simulink model "MMC_phase_discentralized_HAAS_20260927"  (R2024b)
settings: Solver=FixedStepDiscrete  StartTime=t_init_sim  StopTime=sim_time  FixedStep=Ts  RelTol=1e-3
values from neighbouring files (symbols this model uses):
  a = 1    [script_MMC_phase_hackathon_NLM_discentralized_HAAS_20260927.m]
  C1low1_active = 1    [script_MMC_phase_hackathon_NLM_discentralized_HAAS_20260927.m]
  C2low1_active = 1    [script_MMC_phase_hackathon_NLM_discentralized_HAAS_20260927.m]
  C_bus = 4400e-6    (= 0.0044)    [script_MMC_phase_hackathon_NLM_discentralized_HAAS_20260927.m]
  C_M_extra = C_m-twist_high_side_C    [script_MMC_phase_hackathon_NLM_discentralized_HAAS_20260927.m]
  duty_cycle = 1.0    (= 1)    [script_MMC_phase_hackathon_NLM_discentralized_HAAS_20260927.m]
  f0 = 50    [script_MMC_phase_hackathon_NLM_discentralized_HAAS_20260927.m]
  feeder_current_lower_rate_limit = -10    [script_MMC_phase_hackathon_NLM_discentralized_HAAS_20260927.m]    (also in twist_parameters.m = -500)
  feeder_current_tab = [0.328 0.217 0.162 0.132 0.109 0.094 0.083 0.075 0.068 0.062 0.058 0.054 ... (42 elements, 14x3)]    [feeder_current.mat]
  feeder_current_upper_rate_limit = 0.386/(20e-3)    (= 19.3)    [twist_parameters.m]
  is6VExternallySupplied = true    [script_MMC_phase_hackathon_NLM_discentralized_HAAS_20260927.m]
  isFeederJumperOpen = true    [script_MMC_phase_hackathon_NLM_discentralized_HAAS_20260927.m]
  L_arm = 30e-3    (= 0.03)    [script_MMC_phase_hackathon_NLM_discentralized_HAAS_20260927.m]
  m = 1    [script_MMC_phase_hackathon_NLM_discentralized_HAAS_20260927.m]
  N = 5    [script_MMC_phase_hackathon_NLM_discentralized_HAAS_20260927.m]
  power_losses = false    [script_MMC_phase_hackathon_NLM_discentralized_HAAS_20260927.m]
  R = 15    [script_MMC_phase_hackathon_NLM_discentralized_HAAS_20260927.m]
  R_arm = 0.2    [script_MMC_phase_hackathon_NLM_discentralized_HAAS_20260927.m]
  source_V = 0    [script_MMC_phase_hackathon_NLM_discentralized_HAAS_20260927.m]
  Tcom_sample = round(Tcom / Ts)    [script_MMC_phase_hackathon_NLM_discentralized_HAAS_20260927.m]
  time_charge = 0.1    [script_MMC_phase_hackathon_NLM_discentralized_HAAS_20260927.m]
  time_decharge = 1.5    [script_MMC_phase_hackathon_NLM_discentralized_HAAS_20260927.m]
  Ts = 1e-6    (= 1e-06)    [script_MMC_phase_hackathon_NLM_discentralized_HAAS_20260927.m]
  twist_data_acquisition_delay = 50e-9    (= 5e-08)    [script_MMC_phase_hackathon_NLM_discentralized_HAAS_20260927.m]    (also in twist_parameters.m)
  twist_data_sampling_period = 1/twist_freq_data_sampling    (= 5e-05)    [script_MMC_phase_hackathon_NLM_discentralized_HAAS_20260927.m]    (also in twist_parameters.m)
  twist_dead_time = 200e-9    (= 2e-07)    [twist_parameters.m]
  twist_freq_switching = 200e3    (= 200000)    [twist_parameters.m]
  twist_high_side_adc_R = 1/(1/2e6 + 1/2e6 + 1/(330e3+5.6e3))    (= 251272.836178)    [twist_parameters.m]
  twist_high_side_C = 33e-6*4 + 4.7e-6*12    (= 0.0001884)    [twist_parameters.m]
  twist_high_side_feeder_R = 47e3+4.7e3    (= 51700)    [twist_parameters.m]
  twist_high_side_rC = 0.1    [twist_parameters.m]
  twist_low_side_adc_R = 150e3+470    (= 150470)    [twist_parameters.m]
  twist_low_side_C_ceramic = 3*4.7e-6    (= 1.41e-05)    [twist_parameters.m]
  twist_low_side_C_electrolytic = 47e-6    (= 4.7e-05)    [twist_parameters.m]
  twist_low_side_L = 33e-6    (= 3.3e-05)    [twist_parameters.m]
  twist_low_side_rC = 700e-3    (= 0.7)    [twist_parameters.m]
  twist_low_side_rL = 20e-3    (= 0.02)    [twist_parameters.m]
  twist_R_VCC = (tau_VCC/twist_high_side_C  - twist_high_side_rC)/(1-(tau_VCC/twist_high_side_C - twist_high_side_rC)/R_parallel)    (= 1110.74997822)    [twist_parameters.m]
  VDC = 48    [script_MMC_phase_hackathon_NLM_discentralized_HAAS_20260927.m]
undefined symbols (not defined in the file or in its folder): C_SM, feeder_current, gcbh, sps_rtmsupport, twist_low_side_lC
libraries: spsSeriesRLCBranchLib x135, spsTriangleGeneratorLib x60, spsMosfetLib x60, spsCurrentMeasurementLib x43, spsVoltageMeasurementLib x35, spsControlledCurrentSourceLib x30, spsDiodeLib x22, spsIdealSwitchLib x20, spsControlledVoltageSourceLib x1, spsGroundLib x1, spspowerguiLib x1
(part 2 of 22)

== system MMC_phase_discentralized_HAAS_20260927/ /Communication_subsystem/Lower_arm ==
  sync : Inport
  lower_arm_info : Inport  Port=2
  M6_RX_signal : Inport  Port=3
  M7_RX_signal : Inport  Port=4
  M8_RX_signal : Inport  Port=5
  M9_RX_signal : Inport  Port=6
  M10_RX_signal : Inport  Port=7
  M1_Comm : Subsystem
      settings: PortSchema="{\"entries\":[{\"content\":{\"sides\":[{\"content\":{\"connectorIds\":[\"In1\",\"Out2\"]},\"type\":\"ConnectorPlacement.EquallySpacedRectSide\",\"uuid\":\"47077a1e-eba1-4129-8203-93262b2de465\"},{\"content\":{\"connectorIds\":[\"Out1\",\"In3\"],\"side\":\"RIGHT\"},\"type\":\"ConnectorPlacement.EquallySpacedRectSide\",\"uuid\":\"701fdbad-c928-45f3-8ba2-a14f680316f8\"},{\"content\":{\"side\":\"TOP\"},\"type\":\"ConnectorPlacement.EquallySpacedRectSide\",\"uuid\":\"d648951b-caea-4569-a411-8455254fdbc0\"},{\"content\":{\"connectorIds\":[\"In2\"],\"side\":\"BOTTOM\"},\"type\":\"ConnectorPlacement.EquallySpacedRectSide\",\"uuid\":\"07eb9aa1-f407-41f0-8942-d6ed405114b5\"}]},\"type\":\"ConnectorPlacement.EquallySpacedConnector\",\"uuid\":\"7c33ff72-602e-419f-9c2d-5eefc0d60400\"}],\"packageUris\":[\"http://schema.mathworks.com/mf0/Connector/R2020b\"],\"version\":\"1.0\"}"
  M2_Comm : Subsystem
      settings: PortSchema="{\"entries\":[{\"content\":{\"sides\":[{\"content\":{\"connectorIds\":[\"In1\",\"Out2\"]},\"type\":\"ConnectorPlacement.EquallySpacedRectSide\",\"uuid\":\"47077a1e-eba1-4129-8203-93262b2de465\"},{\"content\":{\"connectorIds\":[\"Out1\",\"In3\"],\"side\":\"RIGHT\"},\"type\":\"ConnectorPlacement.EquallySpacedRectSide\",\"uuid\":\"701fdbad-c928-45f3-8ba2-a14f680316f8\"},{\"content\":{\"side\":\"TOP\"},\"type\":\"ConnectorPlacement.EquallySpacedRectSide\",\"uuid\":\"d648951b-caea-4569-a411-8455254fdbc0\"},{\"content\":{\"connectorIds\":[\"In2\"],\"side\":\"BOTTOM\"},\"type\":\"ConnectorPlacement.EquallySpacedRectSide\",\"uuid\":\"01601a56-4c3c-4c18-be21-822f443ca232\"}]},\"type\":\"ConnectorPlacement.EquallySpacedConnector\",\"uuid\":\"7c33ff72-602e-419f-9c2d-5eefc0d60400\"}],\"packageUris\":[\"http://schema.mathworks.com/mf0/Connector/R2020b\"],\"version\":\"1.0\"}"
  M3_Comm : Subsystem
      settings: PortSchema="{\"entries\":[{\"content\":{\"sides\":[{\"content\":{\"connectorIds\":[\"In1\",\"Out2\"]},\"type\":\"ConnectorPlacement.EquallySpacedRectSide\",\"uuid\":\"47077a1e-eba1-4129-8203-93262b2de465\"},{\"content\":{\"connectorIds\":[\"Out1\",\"In3\"],\"side\":\"RIGHT\"},\"type\":\"ConnectorPlacement.EquallySpacedRectSide\",\"uuid\":\"701fdbad-c928-45f3-8ba2-a14f680316f8\"},{\"content\":{\"side\":\"TOP\"},\"type\":\"ConnectorPlacement.EquallySpacedRectSide\",\"uuid\":\"d648951b-caea-4569-a411-8455254fdbc0\"},{\"content\":{\"connectorIds\":[\"In2\"],\"side\":\"BOTTOM\"},\"type\":\"ConnectorPlacement.EquallySpacedRectSide\",\"uuid\":\"b7518228-bb66-4696-b5d4-126a1140e1c3\"}]},\"type\":\"ConnectorPlacement.EquallySpacedConnector\",\"uuid\":\"7c33ff72-602e-419f-9c2d-5eefc0d60400\"}],\"packageUris\":[\"http://schema.mathworks.com/mf0/Connector/R2020b\"],\"version\":\"1.0\"}"
  M4_Comm : Subsystem
      settings: PortSchema="{\"entries\":[{\"content\":{\"sides\":[{\"content\":{\"connectorIds\":[\"In1\",\"Out2\"]},\"type\":\"ConnectorPlacement.EquallySpacedRectSide\",\"uuid\":\"47077a1e-eba1-4129-8203-93262b2de465\"},{\"content\":{\"connectorIds\":[\"Out1\",\"In3\"],\"side\":\"RIGHT\"},\"type\":\"ConnectorPlacement.EquallySpacedRectSide\",\"uuid\":\"701fdbad-c928-45f3-8ba2-a14f680316f8\"},{\"content\":{\"side\":\"TOP\"},\"type\":\"ConnectorPlacement.EquallySpacedRectSide\",\"uuid\":\"d648951b-caea-4569-a411-8455254fdbc0\"},{\"content\":{\"connectorIds\":[\"In2\"],\"side\":\"BOTTOM\"},\"type\":\"ConnectorPlacement.EquallySpacedRectSide\",\"uuid\":\"5f4b38d1-ea61-4297-b8b6-4cb7ffcc6410\"}]},\"type\":\"ConnectorPlacement.EquallySpacedConnector\",\"uuid\":\"7c33ff72-602e-419f-9c2d-5eefc0d60400\"}],\"packageUris\":[\"http://schema.mathworks.com/mf0/Connector/R2020b\"],\"version\":\"1.0\"}"
  M5_Comm : Subsystem
      settings: PortSchema="{\"entries\":[{\"content\":{\"sides\":[{\"content\":{\"connectorIds\":[\"In1\",\"Out2\"]},\"type\":\"ConnectorPlacement.EquallySpacedRectSide\",\"uuid\":\"47077a1e-eba1-4129-8203-93262b2de465\"},{\"content\":{\"connectorIds\":[\"Out1\",\"In3\"],\"side\":\"RIGHT\"},\"type\":\"ConnectorPlacement.EquallySpacedRectSide\",\"uuid\":\"701fdbad-c928-45f3-8ba2-a14f680316f8\"},{\"content\":{\"side\":\"TOP\"},\"type\":\"ConnectorPlacement.EquallySpacedRectSide\",\"uuid\":\"d648951b-caea-4569-a411-8455254fdbc0\"},{\"content\":{\"connectorIds\":[\"In2\"],\"side\":\"BOTTOM\"},\"type\":\"ConnectorPlacement.EquallySpacedRectSide\",\"uuid\":\"cd08f752-2006-4da0-88d6-bb4b20ac3ab7\"}]},\"type\":\"ConnectorPlacement.EquallySpacedConnector\",\"uuid\":\"7c33ff72-602e-419f-9c2d-5eefc0d60400\"}],\"packageUris\":[\"http://schema.mathworks.com/mf0/Connector/R2020b\"],\"version\":\"1.0\"}"
  M6_TX_signal : Outport
  M7_TX_signal : Outport  Port=2
  M8_TX_signal : Outport  Port=3
  M9_TX_signal : Outport  Port=4
  M10_TX_signal : Outport  Port=5
  wires:
  [lower_arm_info] -> M5_Comm/1(TX_variables)
  M4_Comm/1(TX_signal) -> M9_TX_signal/1
  [lower_arm_info] -> M1_Comm/1(TX_variables)
  [lower_arm_info] -> M4_Comm/1(TX_variables)
  M3_Comm/1(TX_signal) -> M8_TX_signal/1
  M2_Comm/1(TX_signal) -> M7_TX_signal/1
  [lower_arm_info] -> M2_Comm/1(TX_variables)
  [lower_arm_info] -> M3_Comm/1(TX_variables)
  M6_RX_signal/1 -> M1_Comm/3(RX_signal)
  [sync] -> M3_Comm/2(sync)
  M8_RX_signal/1 -> M3_Comm/3(RX_signal)
  [sync] -> M5_Comm/2(sync)
  [sync] -> M4_Comm/2(sync)
  [sync] -> M1_Comm/2(sync)
  M10_RX_signal/1 -> M5_Comm/3(RX_signal)
  M1_Comm/1(TX_signal) -> M6_TX_signal/1
  M7_RX_signal/1 -> M2_Comm/3(RX_signal)
  [sync] -> M2_Comm/2(sync)
  M5_Comm/1(TX_signal) -> M10_TX_signal/1
  M9_RX_signal/1 -> M4_Comm/3(RX_signal)
  lower_arm_info/1 -> [lower_arm_info]
  sync/1 -> [sync]

== system MMC_phase_discentralized_HAAS_20260927/ /Communication_subsystem/Upper_arm ==
  upper_arm_info : Inport
  sync : Inport  Port=2
  M1_RX_signal : Inport  Port=3
  M2_RX_signal : Inport  Port=4
  M3_RX_signal : Inport  Port=5
  M4_RX_signal : Inport  Port=6
  M5_RX_signal : Inport  Port=7
  M1_Comm : Subsystem
      settings: PortSchema="{\"entries\":[{\"content\":{\"sides\":[{\"content\":{\"connectorIds\":[\"In1\",\"Out2\"]},\"type\":\"ConnectorPlacement.EquallySpacedRectSide\",\"uuid\":\"c3733cfa-9814-4ae5-a55a-8e5b6f8a57d7\"},{\"content\":{\"connectorIds\":[\"Out1\",\"In3\"],\"side\":\"RIGHT\"},\"type\":\"ConnectorPlacement.EquallySpacedRectSide\",\"uuid\":\"d16535d3-81ee-4162-a646-15cef1f1639a\"},{\"content\":{\"side\":\"TOP\"},\"type\":\"ConnectorPlacement.EquallySpacedRectSide\",\"uuid\":\"672d53ef-99b6-4fa6-8351-42251f607454\"},{\"content\":{\"connectorIds\":[\"In2\"],\"side\":\"BOTTOM\"},\"type\":\"ConnectorPlacement.EquallySpacedRectSide\",\"uuid\":\"a9bd7512-44c2-4af9-8132-4c17be33b3c2\"}]},\"type\":\"ConnectorPlacement.EquallySpacedConnector\",\"uuid\":\"554aea8b-7fd0-4035-ac75-3acab423d605\"}],\"packageUris\":[\"http://schema.mathworks.com/mf0/Connector/R2020b\"],\"version\":\"1.0\"}"
  M2_Comm : Subsystem
      settings: PortSchema="{\"entries\":[{\"content\":{\"sides\":[{\"content\":{\"connectorIds\":[\"In1\",\"Out2\"]},\"type\":\"ConnectorPlacement.EquallySpacedRectSide\",\"uuid\":\"47077a1e-eba1-4129-8203-93262b2de465\"},{\"content\":{\"connectorIds\":[\"Out1\",\"In3\"],\"side\":\"RIGHT\"},\"type\":\"ConnectorPlacement.EquallySpacedRectSide\",\"uuid\":\"701fdbad-c928-45f3-8ba2-a14f680316f8\"},{\"content\":{\"side\":\"TOP\"},\"type\":\"ConnectorPlacement.EquallySpacedRectSide\",\"uuid\":\"d648951b-caea-4569-a411-8455254fdbc0\"},{\"content\":{\"connectorIds\":[\"In2\"],\"side\":\"BOTTOM\"},\"type\":\"ConnectorPlacement.EquallySpacedRectSide\",\"uuid\":\"d4b1d2d6-b4a1-4e2c-9ca6-248db102ef7c\"}]},\"type\":\"ConnectorPlacement.EquallySpacedConnector\",\"uuid\":\"7c33ff72-602e-419f-9c2d-5eefc0d60400\"}],\"packageUris\":[\"http://schema.mathworks.com/mf0/Connector/R2020b\"],\"version\":\"1.0\"}"
  M3_Comm : Subsystem
      settings: PortSchema="{\"entries\":[{\"content\":{\"sides\":[{\"content\":{\"connectorIds\":[\"In1\",\"Out2\"]},\"type\":\"ConnectorPlacement.EquallySpacedRectSide\",\"uuid\":\"47077a1e-eba1-4129-8203-93262b2de465\"},{\"content\":{\"connectorIds\":[\"Out1\",\"In3\"],\"side\":\"RIGHT\"},\"type\":\"ConnectorPlacement.EquallySpacedRectSide\",\"uuid\":\"701fdbad-c928-45f3-8ba2-a14f680316f8\"},{\"content\":{\"side\":\"TOP\"},\"type\":\"ConnectorPlacement.EquallySpacedRectSide\",\"uuid\":\"d648951b-caea-4569-a411-8455254fdbc0\"},{\"content\":{\"connectorIds\":[\"In2\"],\"side\":\"BOTTOM\"},\"type\":\"ConnectorPlacement.EquallySpacedRectSide\",\"uuid\":\"e45915a7-b7a2-4a5e-b9ff-be90cdaaaa95\"}]},\"type\":\"ConnectorPlacement.EquallySpacedConnector\",\"uuid\":\"7c33ff72-602e-419f-9c2d-5eefc0d60400\"}],\"packageUris\":[\"http://schema.mathworks.com/mf0/Connector/R2020b\"],\"version\":\"1.0\"}"
  M4_Comm : Subsystem
      settings: PortSchema="{\"entries\":[{\"content\":{\"sides\":[{\"content\":{\"connectorIds\":[\"In1\",\"Out2\"]},\"type\":\"ConnectorPlacement.EquallySpacedRectSide\",\"uuid\":\"47077a1e-eba1-4129-8203-93262b2de465\"},{\"content\":{\"connectorIds\":[\"Out1\",\"In3\"],\"side\":\"RIGHT\"},\"type\":\"ConnectorPlacement.EquallySpacedRectSide\",\"uuid\":\"701fdbad-c928-45f3-8ba2-a14f680316f8\"},{\"content\":{\"side\":\"TOP\"},\"type\":\"ConnectorPlacement.EquallySpacedRectSide\",\"uuid\":\"d648951b-caea-4569-a411-8455254fdbc0\"},{\"content\":{\"connectorIds\":[\"In2\"],\"side\":\"BOTTOM\"},\"type\":\"ConnectorPlacement.EquallySpacedRectSide\",\"uuid\":\"fe4854bf-7531-4052-9f9a-05b48e3d1945\"}]},\"type\":\"ConnectorPlacement.EquallySpacedConnector\",\"uuid\":\"7c33ff72-602e-419f-9c2d-5eefc0d60400\"}],\"packageUris\":[\"http://schema.mathworks.com/mf0/Connector/R2020b\"],\"version\":\"1.0\"}"
  M5_Comm : Subsystem
      settings: PortSchema="{\"entries\":[{\"content\":{\"sides\":[{\"content\":{\"connectorIds\":[\"In1\",\"Out2\"]},\"type\":\"ConnectorPlacement.EquallySpacedRectSide\",\"uuid\":\"47077a1e-eba1-4129-8203-93262b2de465\"},{\"content\":{\"connectorIds\":[\"Out1\",\"In3\"],\"side\":\"RIGHT\"},\"type\":\"ConnectorPlacement.EquallySpacedRectSide\",\"uuid\":\"701fdbad-c928-45f3-8ba2-a14f680316f8\"},{\"content\":{\"side\":\"TOP\"},\"type\":\"ConnectorPlacement.EquallySpacedRectSide\",\"uuid\":\"d648951b-caea-4569-a411-8455254fdbc0\"},{\"content\":{\"connectorIds\":[\"In2\"],\"side\":\"BOTTOM\"},\"type\":\"ConnectorPlacement.EquallySpacedRectSide\",\"uuid\":\"76d1056e-e7b2-4023-89b8-57825a028de1\"}]},\"type\":\"ConnectorPlacement.EquallySpacedConnector\",\"uuid\":\"7c33ff72-602e-419f-9c2d-5eefc0d60400\"}],\"packageUris\":[\"http://schema.mathworks.com/mf0/Connector/R2020b\"],\"version\":\"1.0\"}"
  M1_TX_signal : Outport
  M2_TX_signal : Outport  Port=2
  M3_TX_signal : Outport  Port=3
  M4_TX_signal : Outport  Port=4
  M5_TX_signal : Outport  Port=5
  RX_Variables : Outport  Port=6
  wires:
  [upper_arm_info] -> M5_Comm/1(TX_variables)
  M4_Comm/1(TX_signal) -> M4_TX_signal/1
  [upper_arm_info] -> M1_Comm/1(TX_variables)
  [upper_arm_info] -> M4_Comm/1(TX_variables)
  M3_Comm/1(TX_signal) -> M3_TX_signal/1
  M2_Comm/1(TX_signal) -> M2_TX_signal/1
  [upper_arm_info] -> M2_Comm/1(TX_variables)
  [upper_arm_info] -> M3_Comm/1(TX_variables)
  M1_RX_signal/1 -> M1_Comm/3(RX_signal)
  [sync] -> M3_Comm/2(sync)
  M3_RX_signal/1 -> M3_Comm/3(RX_signal)
  [sync] -> M5_Comm/2(sync)
  [sync] -> M4_Comm/2(sync)
  [sync] -> M1_Comm/2(sync)
  M5_RX_signal/1 -> M5_Comm/3(RX_signal)
  M1_Comm/1(TX_signal) -> M1_TX_signal/1
  M2_RX_signal/1 -> M2_Comm/3(RX_signal)
  [sync] -> M2_Comm/2(sync)
  M5_Comm/1(TX_signal) -> M5_TX_signal/1
  M4_RX_signal/1 -> M4_Comm/3(RX_signal)
  upper_arm_info/1 -> [upper_arm_info]
  sync/1 -> [sync]
  M1_Comm/2(RX_Variables) -> RX_Variables/1

== system MMC_phase_discentralized_HAAS_20260927/ /Sinus Modulation + Sorting Algorithm/M1 MCU ==
  note: NLM
  note: NLM
  note: Modulation reference
  note: NLM modulation
  Vc_unitaire_stack : Inport
  i_stack : Inport  Port=2
  M_number : Inport  Port=3
  Pulse : Inport  Port=4
  CVB : MATLAB Function  TreatAsAtomicUnit=on
  Constant : Constant  Value=duty_cycle
  Constant4 : Constant  Value=a*1/2
  Gain : Gain  Gain=N
  Gain1 : Gain  Gain=m*1/2
  Gain2 : Gain  Gain=N
  Quantizer : Quantizer  QuantizationInterval=1
  Quantizer1 : Quantizer  QuantizationInterval=1
  Saturation : Saturate  UpperLimit=N  LowerLimit=0
  Saturation1 : Saturate  UpperLimit=N  LowerLimit=0
  Scope : Scope  NumInputPorts=5
  Sine Wave : Sin  Frequency=2*pi*f0  SampleTime=Ts
  Sorting : Subsystem
  Sum1 : Sum  Inputs=|+-
  Sum2 : Sum  Inputs=|++
  g_unitaire_stack : Outport
  N_u : Outport  Port=2
  N_l : Outport  Port=3
  tag scope: ml=global, mu=global
  wires:
  Vc_unitaire_stack/1 -> Sorting/1(Vc_u), Scope/1
  Sorting/1(Ordre_u) -> CVB/1(ordre)
  Saturation/1 -> N_u/1, Scope/4, CVB/3(N_on)
  i_stack/1 -> Scope/2, Sorting/2(i_u)
  Sorting/2(Sens_u) -> CVB/2(sens)
  Pulse/1 -> Scope/5, Sorting/Enable
  CVB/1(y) -> Scope/3, g_unitaire_stack/1
  Constant/1 -> CVB/4(duty_cycle)
  M_number/1 -> CVB/5(M_number)
  Gain/1 -> Quantizer/1
  Gain2/1 -> Quantizer1/1
  Constant4/1 -> Sum2/1, Sum1/1
  Gain1/1 -> Sum1/2, Sum2/2
  Sine Wave/1 -> Gain1/1
  Saturation1/1 -> N_l/1
  Quantizer1/1 -> Saturation1/1
  Sum1/1 -> Gain/1, [mu]
  Quantizer/1 -> Saturation/1
  Sum2/1 -> [ml], Gain2/1

== system MMC_phase_discentralized_HAAS_20260927/ /Sinus Modulation + Sorting Algorithm/M10 MCU ==
  Vc_unitaire_stack : Inport
  i_stack : Inport  Port=2
  N_on_stack : Inport  Port=3
  M_number : Inport  Port=4
  Pulse : Inport  Port=5
  CVB : MATLAB Function  TreatAsAtomicUnit=on
  Constant : Constant  Value=duty_cycle
  Scope : Scope  NumInputPorts=5
  Sorting : Subsystem
  g_unitaire_stack : Outport
  wires:
  Vc_unitaire_stack/1 -> Sorting/1(Vc_u), Scope/1
  Sorting/1(Ordre_u) -> CVB/1(ordre)
  N_on_stack/1 -> Scope/4, CVB/3(N_on)
  i_stack/1 -> Scope/2, Sorting/2(i_u)
  Sorting/2(Sens_u) -> CVB/2(sens)
  Pulse/1 -> Scope/5, Sorting/Enable
  CVB/1(y) -> Scope/3, g_unitaire_stack/1
  Constant/1 -> CVB/4(duty_cycle)
  M_number/1 -> CVB/5(M_number)

== system MMC_phase_discentralized_HAAS_20260927/ /Sinus Modulation + Sorting Algorithm/M2 MCU ==
  Vc_unitaire_stack : Inport
  i_stack : Inport  Port=2
  N_on_stack : Inport  Port=3
  M_number : Inport  Port=4
  Pulse : Inport  Port=5
  CVB : MATLAB Function  TreatAsAtomicUnit=on
  Constant : Constant  Value=duty_cycle
  Scope : Scope  NumInputPorts=5
  Sorting : Subsystem
  g_unitaire_stack : Outport
  wires:
  Vc_unitaire_stack/1 -> Sorting/1(Vc_u), Scope/1
  Sorting/1(Ordre_u) -> CVB/1(ordre)
  N_on_stack/1 -> Scope/4, CVB/3(N_on)
  i_stack/1 -> Scope/2, Sorting/2(i_u)
  Sorting/2(Sens_u) -> CVB/2(sens)
  Pulse/1 -> Scope/5, Sorting/Enable
  CVB/1(y) -> Scope/3, g_unitaire_stack/1
  Constant/1 -> CVB/4(duty_cycle)
  M_number/1 -> CVB/5(M_number)

== system MMC_phase_discentralized_HAAS_20260927/ /Sinus Modulation + Sorting Algorithm/M3 MCU ==
  Vc_unitaire_stack : Inport
  i_stack : Inport  Port=2
  N_on_stack : Inport  Port=3
  M_number : Inport  Port=4
  Pulse : Inport  Port=5
  CVB : MATLAB Function  TreatAsAtomicUnit=on
  Constant : Constant  Value=duty_cycle
  Scope : Scope  NumInputPorts=5
  Sorting : Subsystem
  g_unitaire_stack : Outport
  wires:
  Vc_unitaire_stack/1 -> Sorting/1(Vc_u), Scope/1
  Sorting/1(Ordre_u) -> CVB/1(ordre)
  N_on_stack/1 -> Scope/4, CVB/3(N_on)
  i_stack/1 -> Scope/2, Sorting/2(i_u)
  Sorting/2(Sens_u) -> CVB/2(sens)
  Pulse/1 -> Scope/5, Sorting/Enable
  CVB/1(y) -> Scope/3, g_unitaire_stack/1
  Constant/1 -> CVB/4(duty_cycle)
  M_number/1 -> CVB/5(M_number)

== system MMC_phase_discentralized_HAAS_20260927/ /Sinus Modulation + Sorting Algorithm/M4 MCU ==
  Vc_unitaire_stack : Inport
  i_stack : Inport  Port=2
  N_on_stack : Inport  Port=3
  M_number : Inport  Port=4
  Pulse : Inport  Port=5
  CVB : MATLAB Function  TreatAsAtomicUnit=on
  Constant : Constant  Value=duty_cycle
  Scope : Scope  NumInputPorts=5
  Sorting : Subsystem
  g_unitaire_stack : Outport
  wires:
  Vc_unitaire_stack/1 -> Sorting/1(Vc_u), Scope/1
  Sorting/1(Ordre_u) -> CVB/1(ordre)
  N_on_stack/1 -> Scope/4, CVB/3(N_on)
  i_stack/1 -> Scope/2, Sorting/2(i_u)
  Sorting/2(Sens_u) -> CVB/2(sens)
  Pulse/1 -> Scope/5, Sorting/Enable
  CVB/1(y) -> Scope/3, g_unitaire_stack/1
  Constant/1 -> CVB/4(duty_cycle)
  M_number/1 -> CVB/5(M_number)

== system MMC_phase_discentralized_HAAS_20260927/ /Sinus Modulation + Sorting Algorithm/M5 MCU ==
  Vc_unitaire_stack : Inport
  i_stack : Inport  Port=2
  N_on_stack : Inport  Port=3
  M_number : Inport  Port=4
  Pulse : Inport  Port=5
  CVB : MATLAB Function  TreatAsAtomicUnit=on
  Constant : Constant  Value=duty_cycle
  Scope : Scope  NumInputPorts=5
  Sorting : Subsystem
  g_unitaire_stack : Outport
  wires:
  Vc_unitaire_stack/1 -> Sorting/1(Vc_u), Scope/1
  Sorting/1(Ordre_u) -> CVB/1(ordre)
  N_on_stack/1 -> Scope/4, CVB/3(N_on)
  i_stack/1 -> Scope/2, Sorting/2(i_u)
  Sorting/2(Sens_u) -> CVB/2(sens)
  Pulse/1 -> Scope/5, Sorting/Enable
  CVB/1(y) -> Scope/3, g_unitaire_stack/1
  Constant/1 -> CVB/4(duty_cycle)
  M_number/1 -> CVB/5(M_number)

== system MMC_phase_discentralized_HAAS_20260927/ /Sinus Modulation + Sorting Algorithm/M6 MCU ==
  Vc_unitaire_stack : Inport
  i_stack : Inport  Port=2
  N_on_stack : Inport  Port=3
  M_number : Inport  Port=4
  Pulse : Inport  Port=5
  CVB : MATLAB Function  TreatAsAtomicUnit=on
  Constant : Constant  Value=duty_cycle
  Scope : Scope  NumInputPorts=5
  Sorting : Subsystem
  g_unitaire_stack : Outport
  wires:
  Vc_unitaire_stack/1 -> Sorting/1(Vc_u), Scope/1
  Sorting/1(Ordre_u) -> CVB/1(ordre)
  N_on_stack/1 -> Scope/4, CVB/3(N_on)
  i_stack/1 -> Scope/2, Sorting/2(i_u)
  Sorting/2(Sens_u) -> CVB/2(sens)
  Pulse/1 -> Scope/5, Sorting/Enable
  CVB/1(y) -> Scope/3, g_unitaire_stack/1
  Constant/1 -> CVB/4(duty_cycle)
  M_number/1 -> CVB/5(M_number)

== system MMC_phase_discentralized_HAAS_20260927/ /Sinus Modulation + Sorting Algorithm/M7 MCU ==
  Vc_unitaire_stack : Inport
  i_stack : Inport  Port=2
  N_on_stack : Inport  Port=3
  M_number : Inport  Port=4
  Pulse : Inport  Port=5
  CVB : MATLAB Function  TreatAsAtomicUnit=on
  Constant : Constant  Value=duty_cycle
  Scope : Scope  NumInputPorts=5
  Sorting : Subsystem
  g_unitaire_stack : Outport
  wires:
  Vc_unitaire_stack/1 -> Sorting/1(Vc_u), Scope/1
  Sorting/1(Ordre_u) -> CVB/1(ordre)
  N_on_stack/1 -> Scope/4, CVB/3(N_on)
  i_stack/1 -> Scope/2, Sorting/2(i_u)
  Sorting/2(Sens_u) -> CVB/2(sens)
  Pulse/1 -> Scope/5, Sorting/Enable
  CVB/1(y) -> Scope/3, g_unitaire_stack/1
  Constant/1 -> CVB/4(duty_cycle)
  M_number/1 -> CVB/5(M_number)

== system MMC_phase_discentralized_HAAS_20260927/ /Sinus Modulation + Sorting Algorithm/M8 MCU ==
  Vc_unitaire_stack : Inport
  i_stack : Inport  Port=2
  N_on_stack : Inport  Port=3
  M_number : Inport  Port=4
  Pulse : Inport  Port=5
  CVB : MATLAB Function  TreatAsAtomicUnit=on
  Constant : Constant  Value=duty_cycle
  Scope : Scope  NumInputPorts=5
  Sorting : Subsystem
  g_unitaire_stack : Outport
  wires:
  Vc_unitaire_stack/1 -> Sorting/1(Vc_u), Scope/1
  Sorting/1(Ordre_u) -> CVB/1(ordre)
  N_on_stack/1 -> Scope/4, CVB/3(N_on)
  i_stack/1 -> Scope/2, Sorting/2(i_u)
  Sorting/2(Sens_u) -> CVB/2(sens)
  Pulse/1 -> Scope/5, Sorting/Enable
  CVB/1(y) -> Scope/3, g_unitaire_stack/1
  Constant/1 -> CVB/4(duty_cycle)
  M_number/1 -> CVB/5(M_number)

== system MMC_phase_discentralized_HAAS_20260927/ /Sinus Modulation + Sorting Algorithm/M9 MCU ==
  Vc_unitaire_stack : Inport
  i_stack : Inport  Port=2
  N_on_stack : Inport  Port=3
  M_number : Inport  Port=4
  Pulse : Inport  Port=5
  CVB : MATLAB Function  TreatAsAtomicUnit=on
  Constant : Constant  Value=duty_cycle
  Scope : Scope  NumInputPorts=5
  Sorting : Subsystem
  g_unitaire_stack : Outport
  wires:
  Vc_unitaire_stack/1 -> Sorting/1(Vc_u), Scope/1
  Sorting/1(Ordre_u) -> CVB/1(ordre)
  N_on_stack/1 -> Scope/4, CVB/3(N_on)
  i_stack/1 -> Scope/2, Sorting/2(i_u)
  Sorting/2(Sens_u) -> CVB/2(sens)
  Pulse/1 -> Scope/5, Sorting/Enable
  CVB/1(y) -> Scope/3, g_unitaire_stack/1
  Constant/1 -> CVB/4(duty_cycle)
  M_number/1 -> CVB/5(M_number)

== system MMC_phase_discentralized_HAAS_20260927/ /Subsystem/Subsystem ==
  note: MMC electrical circuit connected to the modules hardware block
  note: MMC electrical circuit connected to the modules hardware block
  note: MMC electrical circuit connected to the modules hardware block
  note: MMC electrical circuit connected to the modules hardware block
  note: MMC electrical circuit connected to the modules hardware block
  duty_cycle_M1 : Inport
  block_M1 : Inport  Port=2
  duty_cycle_M2 : Inport  Port=3
  block_M2 : Inport  Port=4
  duty_cycle_M3 : Inport  Port=5
  block_M3 : Inport  Port=6
  duty_cycle_M4 : Inport  Port=7
  block_M4 : Inport  Port=8
  duty_cycle_M5 : Inport  Port=9
  block_M5 : Inport  Port=10
  AC Load{6..10} (5 alike) : spsSeriesRLCBranchLib/Series RLC Branch  LConnTagsString=__new0  RConnTagsString=__new0  BranchType=C  Resistance=R  Inductance=L_arm  SetiL0=off  InitialCurrent=0  Capacitance=C_M_extra  Setx0=on  InitialVoltage=source_V  Measurements=None
  Hardware M1 : Subsystem
  Hardware M2 : Subsystem
  Hardware M3 : Subsystem
  Hardware M4 : Subsystem
  Hardware M5 : Subsystem
  V1low_M1 : PMIOPort  Side=Left
  Low_GND_M5 : PMIOPort  Port=2  Side=Left
  i_mod_M1 : Outport
  v_cap_M1 : Outport  Port=2
  v_cap_M2 : Outport  Port=3
  v_cap_M3 : Outport  Port=4
  v_cap_M4 : Outport  Port=5
  v_cap_M5 : Outport  Port=6
  wires:
  Hardware M1/1(v_cap) -> v_cap_M1/1
  duty_cycle_M1/1 -> Hardware M1/1(duty_cycle)
  duty_cycle_M2/1 -> Hardware M2/1(duty_cycle)
  block_M5/1 -> Hardware M5/2(block)
  Hardware M3/1(v_cap) -> v_cap_M3/1
  block_M1/1 -> Hardware M1/2(block)
  Hardware M1/2(i_mod) -> i_mod_M1/1
  duty_cycle_M4/1 -> Hardware M4/1(duty_cycle)
  block_M2/1 -> Hardware M2/2(block)
  Hardware M5/1(v_cap) -> v_cap_M5/1
  Hardware M2/1(v_cap) -> v_cap_M2/1
  duty_cycle_M3/1 -> Hardware M3/1(duty_cycle)
  duty_cycle_M5/1 -> Hardware M5/1(duty_cycle)
  block_M4/1 -> Hardware M4/2(block)
  block_M3/1 -> Hardware M3/2(block)
  Hardware M4/1(v_cap) -> v_cap_M4/1
  connections:
  Hardware M5/RConn2 -- AC Load10/RConn1
  AC Load6/LConn1 -- Hardware M1/RConn1
  Hardware M1/LConn2 -- Hardware M2/LConn1
  Hardware M3/LConn2 -- Hardware M4/LConn1
  Hardware M5/RConn1 -- AC Load10/LConn1
  AC Load6/RConn1 -- Hardware M1/RConn2
  Hardware M2/RConn2 -- AC Load7/RConn1
  Hardware M2/LConn2 -- Hardware M3/LConn1
  Hardware M2/RConn1 -- AC Load7/LConn1
  Hardware M3/RConn1 -- AC Load8/LConn1
  Hardware M3/RConn2 -- AC Load8/RConn1
  Hardware M4/RConn2 -- AC Load9/RConn1
  Hardware M4/RConn1 -- AC Load9/LConn1
  Hardware M4/LConn2 -- Hardware M5/LConn1
  V1low_M1/RConn1 -- Hardware M1/LConn1
  Low_GND_M5/RConn1 -- Hardware M5/LConn2

== system MMC_phase_discentralized_HAAS_20260927/ /Subsystem/Subsystem1 ==
  note: MMC electrical circuit connected to the modules hardware block
  note: MMC electrical circuit connected to the modules hardware block
  note: MMC electrical circuit connected to the modules hardware block
  note: MMC electrical circuit connected to the modules hardware block
  note: MMC electrical circuit connected to the modules hardware block
  duty_cycle_M1 : Inport
  block_M1 : Inport  Port=2
  duty_cycle_M2 : Inport  Port=3
  block_M2 : Inport  Port=4
  duty_cycle_M3 : Inport  Port=5
  block_M3 : Inport  Port=6
  duty_cycle_M4 : Inport  Port=7
  block_M4 : Inport  Port=8
  duty_cycle_M5 : Inport  Port=9
  block_M5 : Inport  Port=10
  AC Load{6..10} (5 alike) : spsSeriesRLCBranchLib/Series RLC Branch  LConnTagsString=__new0  RConnTagsString=__new0  BranchType=C  Resistance=R  Inductance=L_arm  SetiL0=off  InitialCurrent=0  Capacitance=C_M_extra  Setx0=on  InitialVoltage=source_V  Measurements=None
  Hardware M1 : Subsystem
  Hardware M2 : Subsystem
  Hardware M3 : Subsystem
  Hardware M4 : Subsystem
  Hardware M5 : Subsystem
  V1low_M1 : PMIOPort  Side=Left
  Low_GND_M5 : PMIOPort  Port=2  Side=Left
  i_mod_M1 : Outport
  v_cap_M1 : Outport  Port=2
  v_cap_M2 : Outport  Port=3
  v_cap_M3 : Outport  Port=4
  v_cap_M4 : Outport  Port=5
  v_cap_M5 : Outport  Port=6
  wires:
  Hardware M1/1(v_cap) -> v_cap_M1/1
  duty_cycle_M1/1 -> Hardware M1/1(duty_cycle)
  duty_cycle_M2/1 -> Hardware M2/1(duty_cycle)
  block_M5/1 -> Hardware M5/2(block)
  Hardware M3/1(v_cap) -> v_cap_M3/1
  block_M1/1 -> Hardware M1/2(block)
  Hardware M1/2(i_mod) -> i_mod_M1/1
  duty_cycle_M4/1 -> Hardware M4/1(duty_cycle)
  block_M2/1 -> Hardware M2/2(block)
  Hardware M5/1(v_cap) -> v_cap_M5/1
  Hardware M2/1(v_cap) -> v_cap_M2/1
  duty_cycle_M3/1 -> Hardware M3/1(duty_cycle)
  duty_cycle_M5/1 -> Hardware M5/1(duty_cycle)
  block_M4/1 -> Hardware M4/2(block)
  block_M3/1 -> Hardware M3/2(block)
  Hardware M4/1(v_cap) -> v_cap_M4/1
  connections:
  Hardware M5/RConn2 -- AC Load10/RConn1
  AC Load6/LConn1 -- Hardware M1/RConn1
  Hardware M1/LConn2 -- Hardware M2/LConn1
  Hardware M3/LConn2 -- Hardware M4/LConn1
  Hardware M5/RConn1 -- AC Load10/LConn1
  AC Load6/RConn1 -- Hardware M1/RConn2
  Hardware M2/RConn2 -- AC Load7/RConn1
  Hardware M2/LConn2 -- Hardware M3/LConn1
  Hardware M2/RConn1 -- AC Load7/LConn1
  Hardware M3/RConn1 -- AC Load8/LConn1
  Hardware M3/RConn2 -- AC Load8/RConn1
  Hardware M4/RConn2 -- AC Load9/RConn1
  Hardware M4/RConn1 -- AC Load9/LConn1
  Hardware M4/LConn2 -- Hardware M5/LConn1
  V1low_M1/RConn1 -- Hardware M1/LConn1
  Low_GND_M5/RConn1 -- Hardware M5/LConn2

== system MMC_phase_discentralized_HAAS_20260927/ /Communication_subsystem/Lower_arm/M1_Comm ==
  TX_variables : Inport
  sync : Inport  Port=2
  RX_signal : Inport  Port=3
  Data Type Conversion : DataTypeConversion  OutDataTypeStr=single  SaturateOnIntegerOverflow=off  RndMeth=Floor
  Delay : Delay  DelayLength=Tcom_sample
  Snapshot : MATLAB Function  TreatAsAtomicUnit=on
  TxFormatter : MATLAB Function  TreatAsAtomicUnit=on
  node_id : Constant  Value=6
  TX_signal : Outport
  RX_Variables : Outport  Port=2
  wires:
  TX_variables/1 -> Data Type Conversion/1
  RX_signal/1 -> Snapshot/1(rx_signal), TxFormatter/3(rx_signal)
  TxFormatter/1(tx_data) -> Delay/1
  Data Type Conversion/1 -> TxFormatter/1(tx_variables)
  Snapshot/1(rx_variables) -> RX_Variables/1
  sync/1 -> Snapshot/3(sync), TxFormatter/2(sync)
  node_id/1 -> TxFormatter/4(node_id)
  Delay/1 -> TX_signal/1

== system MMC_phase_discentralized_HAAS_20260927/ /Communication_subsystem/Lower_arm/M2_Comm ==
  TX_variables : Inport
  sync : Inport  Port=2
  RX_signal : Inport  Port=3
  Data Type Conversion : DataTypeConversion  OutDataTypeStr=single  SaturateOnIntegerOverflow=off  RndMeth=Floor
  Delay : Delay  DelayLength=Tcom_sample
  Snapshot : MATLAB Function  TreatAsAtomicUnit=on
  TxFormatter : MATLAB Function  TreatAsAtomicUnit=on
  node_id : Constant  Value=7
  TX_signal : Outport
  RX_Variables : Outport  Port=2
  wires:
  TX_variables/1 -> Data Type Conversion/1
  RX_signal/1 -> Snapshot/1(rx_signal), TxFormatter/3(rx_signal)
  TxFormatter/1(tx_data) -> Delay/1
  Data Type Conversion/1 -> TxFormatter/1(tx_variables)
  Snapshot/1(rx_variables) -> RX_Variables/1
  sync/1 -> Snapshot/3(sync), TxFormatter/2(sync)
  node_id/1 -> TxFormatter/4(node_id)
  Delay/1 -> TX_signal/1

== system MMC_phase_discentralized_HAAS_20260927/ /Communication_subsystem/Lower_arm/M3_Comm ==
  TX_variables : Inport
  sync : Inport  Port=2
  RX_signal : Inport  Port=3
  Data Type Conversion : DataTypeConversion  OutDataTypeStr=single  SaturateOnIntegerOverflow=off  RndMeth=Floor
  Delay : Delay  DelayLength=Tcom_sample
  Snapshot : MATLAB Function  TreatAsAtomicUnit=on
  TxFormatter : MATLAB Function  TreatAsAtomicUnit=on
  node_id : Constant  Value=8
  TX_signal : Outport
  RX_Variables : Outport  Port=2
  wires:
  TX_variables/1 -> Data Type Conversion/1
  RX_signal/1 -> Snapshot/1(rx_signal), TxFormatter/3(rx_signal)
  TxFormatter/1(tx_data) -> Delay/1
  Data Type Conversion/1 -> TxFormatter/1(tx_variables)
  Snapshot/1(rx_variables) -> RX_Variables/1
  sync/1 -> Snapshot/3(sync), TxFormatter/2(sync)
  node_id/1 -> TxFormatter/4(node_id)
  Delay/1 -> TX_signal/1

== system MMC_phase_discentralized_HAAS_20260927/ /Communication_subsystem/Lower_arm/M4_Comm ==
  TX_variables : Inport
  sync : Inport  Port=2
  RX_signal : Inport  Port=3
  Data Type Conversion : DataTypeConversion  OutDataTypeStr=single  SaturateOnIntegerOverflow=off  RndMeth=Floor
  Delay : Delay  DelayLength=Tcom_sample
  Snapshot : MATLAB Function  TreatAsAtomicUnit=on
  TxFormatter : MATLAB Function  TreatAsAtomicUnit=on
  node_id : Constant  Value=9
  TX_signal : Outport
  RX_Variables : Outport  Port=2
  wires:
  TX_variables/1 -> Data Type Conversion/1
  RX_signal/1 -> Snapshot/1(rx_signal), TxFormatter/3(rx_signal)
  TxFormatter/1(tx_data) -> Delay/1
  Data Type Conversion/1 -> TxFormatter/1(tx_variables)
  Snapshot/1(rx_variables) -> RX_Variables/1
  sync/1 -> Snapshot/3(sync), TxFormatter/2(sync)
  node_id/1 -> TxFormatter/4(node_id)
  Delay/1 -> TX_signal/1

== system MMC_phase_discentralized_HAAS_20260927/ /Communication_subsystem/Lower_arm/M5_Comm ==
  TX_variables : Inport
  sync : Inport  Port=2
  RX_signal : Inport  Port=3
  Data Type Conversion : DataTypeConversion  OutDataTypeStr=single  SaturateOnIntegerOverflow=off  RndMeth=Floor
  Delay : Delay  DelayLength=Tcom_sample
  Snapshot : MATLAB Function  TreatAsAtomicUnit=on
  TxFormatter : MATLAB Function  TreatAsAtomicUnit=on
  node_id : Constant  Value=10
  TX_signal : Outport
  RX_Variables : Outport  Port=2
  wires:
  TX_variables/1 -> Data Type Conversion/1
  RX_signal/1 -> Snapshot/1(rx_signal), TxFormatter/3(rx_signal)
  TxFormatter/1(tx_data) -> Delay/1
  Data Type Conversion/1 -> TxFormatter/1(tx_variables)
  Snapshot/1(rx_variables) -> RX_Variables/1
  sync/1 -> Snapshot/3(sync), TxFormatter/2(sync)
  node_id/1 -> TxFormatter/4(node_id)
  Delay/1 -> TX_signal/1

== system MMC_phase_discentralized_HAAS_20260927/ /Communication_subsystem/Upper_arm/M1_Comm ==
  TX_variables : Inport
  sync : Inport  Port=2
  RX_signal : Inport  Port=3
  Data Type Conversion : DataTypeConversion  OutDataTypeStr=single  SaturateOnIntegerOverflow=off  RndMeth=Floor
  Delay : Delay  DelayLength=Tcom_sample
  Delay1 : Delay  DelayLength=1
  Delay2 : Delay  DelayLength=1
  Scope : Scope  NumInputPorts=6
  Scope1 : Scope  NumInputPorts=2
  Snapshot : MATLAB Function  TreatAsAtomicUnit=on
  TxFormatter : MATLAB Function  TreatAsAtomicUnit=on
  node_id : Constant
  TX_signal : Outport
  RX_Variables : Outport  Port=2
  wires:
  TX_variables/1 -> Data Type Conversion/1
  TxFormatter/1(tx_data) -> Delay/1
  Delay/1 -> TX_signal/1
  sync/1 -> Snapshot/3(sync), Scope1/1, TxFormatter/2(sync)  "Ctrl_task"
  RX_signal/1 -> Snapshot/1(rx_signal), TxFormatter/3(rx_signal)
  Snapshot/1(rx_variables) -> RX_Variables/1
  Data Type Conversion/1 -> TxFormatter/1(tx_variables)
  node_id/1 -> TxFormatter/4(node_id)
  TxFormatter/2(tx_fire) -> Scope/1
  TxFormatter/3(tx_busy) -> Scope/2
  TxFormatter/5(rx_count_dbg) -> Scope/4
  TxFormatter/6(rx_id_dbg) -> Scope1/2, Scope/5  "1 -> 2 data"
  TxFormatter/7(overrun) -> Scope/6
  TxFormatter/8(local_frame_snapshot) -> Delay1/1
  Delay1/1 -> Snapshot/2(local_frame_snapshot)
  TxFormatter/4(round_done) -> Scope/3, Delay2/1
  Delay2/1 -> Snapshot/4(round_done)

== system MMC_phase_discentralized_HAAS_20260927/ /Communication_subsystem/Upper_arm/M2_Comm ==
  TX_variables : Inport
  sync : Inport  Port=2
  RX_signal : Inport  Port=3
  Data Type Conversion : DataTypeConversion  OutDataTypeStr=single  SaturateOnIntegerOverflow=off  RndMeth=Floor
  Delay : Delay  DelayLength=Tcom_sample
  Delay1 : Delay  DelayLength=1
  Scope : Scope  NumInputPorts=6
  Snapshot : MATLAB Function  TreatAsAtomicUnit=on
  TxFormatter : MATLAB Function  TreatAsAtomicUnit=on
  node_id : Constant  Value=2
  TX_signal : Outport
  RX_Variables : Outport  Port=2
  wires:
  TxFormatter/2(tx_fire) -> Scope/1
  TxFormatter/3(tx_busy) -> Scope/2
  TxFormatter/8(local_frame_snapshot) -> Delay1/1
  TxFormatter/7(overrun) -> Scope/6
  TX_variables/1 -> Data Type Conversion/1
  Delay/1 -> TX_signal/1
  TxFormatter/4(round_done) -> Scope/3
  Snapshot/1(rx_variables) -> RX_Variables/1
  TxFormatter/1(tx_data) -> Delay/1
  Delay1/1 -> Snapshot/2(local_frame_snapshot)
  Data Type Conversion/1 -> TxFormatter/1(tx_variables)
  sync/1 -> Snapshot/3(sync), TxFormatter/2(sync)
  node_id/1 -> TxFormatter/4(node_id)
  TxFormatter/6(rx_id_dbg) -> Scope/5
  RX_signal/1 -> Snapshot/1(rx_signal), TxFormatter/3(rx_signal)
  TxFormatter/5(rx_count_dbg) -> Scope/4

== system MMC_phase_discentralized_HAAS_20260927/ /Communication_subsystem/Upper_arm/M3_Comm ==
  TX_variables : Inport
  sync : Inport  Port=2
  RX_signal : Inport  Port=3
  Data Type Conversion : DataTypeConversion  OutDataTypeStr=single  SaturateOnIntegerOverflow=off  RndMeth=Floor
  Delay : Delay  DelayLength=Tcom_sample
  Delay1 : Delay  DelayLength=1
  Scope : Scope  NumInputPorts=6
  Snapshot : MATLAB Function  TreatAsAtomicUnit=on
  TxFormatter : MATLAB Function  TreatAsAtomicUnit=on
  node_id : Constant  Value=3
  TX_signal : Outport
  RX_Variables : Outport  Port=2
  wires:
  TxFormatter/2(tx_fire) -> Scope/1
  TxFormatter/3(tx_busy) -> Scope/2
  TxFormatter/8(local_frame_snapshot) -> Delay1/1
  TxFormatter/7(overrun) -> Scope/6
  TX_variables/1 -> Data Type Conversion/1
  Delay/1 -> TX_signal/1
  TxFormatter/4(round_done) -> Scope/3
  Snapshot/1(rx_variables) -> RX_Variables/1
  TxFormatter/1(tx_data) -> Delay/1
  Delay1/1 -> Snapshot/2(local_frame_snapshot)
  Data Type Conversion/1 -> TxFormatter/1(tx_variables)
  sync/1 -> Snapshot/3(sync), TxFormatter/2(sync)
  node_id/1 -> TxFormatter/4(node_id)
  TxFormatter/6(rx_id_dbg) -> Scope/5
  RX_signal/1 -> Snapshot/1(rx_signal), TxFormatter/3(rx_signal)
  TxFormatter/5(rx_count_dbg) -> Scope/4

== system MMC_phase_discentralized_HAAS_20260927/ /Communication_subsystem/Upper_arm/M4_Comm ==
  TX_variables : Inport
  sync : Inport  Port=2
  RX_signal : Inport  Port=3
  Data Type Conversion : DataTypeConversion  OutDataTypeStr=single  SaturateOnIntegerOverflow=off  RndMeth=Floor
  Delay : Delay  DelayLength=Tcom_sample
  Delay1 : Delay  DelayLength=1
  Scope : Scope  NumInputPorts=6
  Snapshot : MATLAB Function  TreatAsAtomicUnit=on
  TxFormatter : MATLAB Function  TreatAsAtomicUnit=on
  node_id : Constant  Value=4
  TX_signal : Outport
  RX_Variables : Outport  Port=2
  wires:
  TxFormatter/2(tx_fire) -> Scope/1
  TxFormatter/3(tx_busy) -> Scope/2
  TxFormatter/8(local_frame_snapshot) -> Delay1/1
  TxFormatter/7(overrun) -> Scope/6
  TX_variables/1 -> Data Type Conversion/1
  Delay/1 -> TX_signal/1
  TxFormatter/4(round_done) -> Scope/3
  Snapshot/1(rx_variables) -> RX_Variables/1
  TxFormatter/1(tx_data) -> Delay/1
  Delay1/1 -> Snapshot/2(local_frame_snapshot)
  Data Type Conversion/1 -> TxFormatter/1(tx_variables)
  sync/1 -> Snapshot/3(sync), TxFormatter/2(sync)
  node_id/1 -> TxFormatter/4(node_id)
  TxFormatter/6(rx_id_dbg) -> Scope/5
  RX_signal/1 -> Snapshot/1(rx_signal), TxFormatter/3(rx_signal)
  TxFormatter/5(rx_count_dbg) -> Scope/4

== system MMC_phase_discentralized_HAAS_20260927/ /Communication_subsystem/Upper_arm/M5_Comm ==
  TX_variables : Inport
  sync : Inport  Port=2
  RX_signal : Inport  Port=3
  Data Type Conversion : DataTypeConversion  OutDataTypeStr=single  SaturateOnIntegerOverflow=off  RndMeth=Floor
  Delay : Delay  DelayLength=Tcom_sample
  Snapshot : MATLAB Function  TreatAsAtomicUnit=on
  TxFormatter : MATLAB Function  TreatAsAtomicUnit=on
  node_id : Constant  Value=5
  TX_signal : Outport
  RX_Variables : Outport  Port=2
  wires:
  TX_variables/1 -> Data Type Conversion/1
  RX_signal/1 -> Snapshot/1(rx_signal), TxFormatter/3(rx_signal)
  TxFormatter/1(tx_data) -> Delay/1
  Data Type Conversion/1 -> TxFormatter/1(tx_variables)
  Snapshot/1(rx_variables) -> RX_Variables/1
  sync/1 -> Snapshot/3(sync), TxFormatter/2(sync)
  node_id/1 -> TxFormatter/4(node_id)
  Delay/1 -> TX_signal/1

== system MMC_phase_discentralized_HAAS_20260927/ /Sinus Modulation + Sorting Algorithm/M1 MCU/Sorting ==
  Vc_u : Inport
  i_u : Inport  Port=2
  Pulse : EnablePort
  Tri2 : MATLAB Function  TreatAsAtomicUnit=on
  Ordre_u : Outport
  Sens_u : Outport  Port=2
  wires:
  Vc_u/1 -> Tri2/1(Vcp)
  i_u/1 -> Tri2/2(i)
  Tri2/1(ordre) -> Ordre_u/1
  Tri2/2(sens) -> Sens_u/1  "Ordre"

== system MMC_phase_discentralized_HAAS_20260927/ /Sinus Modulation + Sorting Algorithm/M10 MCU/Sorting ==
  Vc_u : Inport
  i_u : Inport  Port=2
  Pulse : EnablePort
  Tri2 : MATLAB Function  TreatAsAtomicUnit=on
  Ordre_u : Outport
  Sens_u : Outport  Port=2
  wires:
  Vc_u/1 -> Tri2/1(Vcp)
  i_u/1 -> Tri2/2(i)
  Tri2/1(ordre) -> Ordre_u/1
  Tri2/2(sens) -> Sens_u/1  "Ordre"

== system MMC_phase_discentralized_HAAS_20260927/ /Sinus Modulation + Sorting Algorithm/M2 MCU/Sorting ==
  Vc_u : Inport
  i_u : Inport  Port=2
  Pulse : EnablePort
  Tri2 : MATLAB Function  TreatAsAtomicUnit=on
  Ordre_u : Outport
  Sens_u : Outport  Port=2
  wires:
  Vc_u/1 -> Tri2/1(Vcp)
  i_u/1 -> Tri2/2(i)
  Tri2/1(ordre) -> Ordre_u/1
  Tri2/2(sens) -> Sens_u/1  "Ordre"

== system MMC_phase_discentralized_HAAS_20260927/ /Sinus Modulation + Sorting Algorithm/M3 MCU/Sorting ==
  Vc_u : Inport
  i_u : Inport  Port=2
  Pulse : EnablePort
  Tri2 : MATLAB Function  TreatAsAtomicUnit=on
  Ordre_u : Outport
  Sens_u : Outport  Port=2
  wires:
  Vc_u/1 -> Tri2/1(Vcp)
  i_u/1 -> Tri2/2(i)
  Tri2/1(ordre) -> Ordre_u/1
  Tri2/2(sens) -> Sens_u/1  "Ordre"

== system MMC_phase_discentralized_HAAS_20260927/ /Sinus Modulation + Sorting Algorithm/M4 MCU/Sorting ==
  Vc_u : Inport
  i_u : Inport  Port=2
  Pulse : EnablePort
  Tri2 : MATLAB Function  TreatAsAtomicUnit=on
  Ordre_u : Outport
  Sens_u : Outport  Port=2
  wires:
  Vc_u/1 -> Tri2/1(Vcp)
  i_u/1 -> Tri2/2(i)
  Tri2/1(ordre) -> Ordre_u/1
  Tri2/2(sens) -> Sens_u/1  "Ordre"

== system MMC_phase_discentralized_HAAS_20260927/ /Sinus Modulation + Sorting Algorithm/M5 MCU/Sorting ==
  Vc_u : Inport
  i_u : Inport  Port=2
  Pulse : EnablePort
  Tri2 : MATLAB Function  TreatAsAtomicUnit=on
  Ordre_u : Outport
  Sens_u : Outport  Port=2
  wires:
  Vc_u/1 -> Tri2/1(Vcp)
  i_u/1 -> Tri2/2(i)
  Tri2/1(ordre) -> Ordre_u/1
  Tri2/2(sens) -> Sens_u/1  "Ordre"

== system MMC_phase_discentralized_HAAS_20260927/ /Sinus Modulation + Sorting Algorithm/M6 MCU/Sorting ==
  Vc_u : Inport
  i_u : Inport  Port=2
  Pulse : EnablePort
  Tri2 : MATLAB Function  TreatAsAtomicUnit=on
  Ordre_u : Outport
  Sens_u : Outport  Port=2
  wires:
  Vc_u/1 -> Tri2/1(Vcp)
  i_u/1 -> Tri2/2(i)
  Tri2/1(ordre) -> Ordre_u/1
  Tri2/2(sens) -> Sens_u/1  "Ordre"

== system MMC_phase_discentralized_HAAS_20260927/ /Sinus Modulation + Sorting Algorithm/M7 MCU/Sorting ==
  Vc_u : Inport
  i_u : Inport  Port=2
  Pulse : EnablePort
  Tri2 : MATLAB Function  TreatAsAtomicUnit=on
  Ordre_u : Outport
  Sens_u : Outport  Port=2
  wires:
  Vc_u/1 -> Tri2/1(Vcp)
  i_u/1 -> Tri2/2(i)
  Tri2/1(ordre) -> Ordre_u/1
  Tri2/2(sens) -> Sens_u/1  "Ordre"

== system MMC_phase_discentralized_HAAS_20260927/ /Sinus Modulation + Sorting Algorithm/M8 MCU/Sorting ==
  Vc_u : Inport
  i_u : Inport  Port=2
  Pulse : EnablePort
  Tri2 : MATLAB Function  TreatAsAtomicUnit=on
  Ordre_u : Outport
  Sens_u : Outport  Port=2
  wires:
  Vc_u/1 -> Tri2/1(Vcp)
  i_u/1 -> Tri2/2(i)
  Tri2/1(ordre) -> Ordre_u/1
  Tri2/2(sens) -> Sens_u/1  "Ordre"

== system MMC_phase_discentralized_HAAS_20260927/ /Sinus Modulation + Sorting Algorithm/M9 MCU/Sorting ==
  Vc_u : Inport
  i_u : Inport  Port=2
  Pulse : EnablePort
  Tri2 : MATLAB Function  TreatAsAtomicUnit=on
  Ordre_u : Outport
  Sens_u : Outport  Port=2
  wires:
  Vc_u/1 -> Tri2/1(Vcp)
  i_u/1 -> Tri2/2(i)
  Tri2/1(ordre) -> Ordre_u/1
  Tri2/2(sens) -> Sens_u/1  "Ordre"
